simulink model "scara_ctc_sim"  (R2024a)
settings: Solver=ode4  StartTime=0.0  StopTime=4.0  FixedStep=0.005  RelTol=1e-3
settings Model: Creator=42962  LastModifiedBy=42962

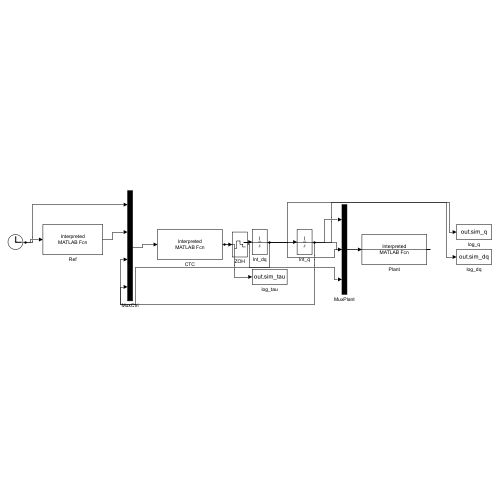
[thumbnail: Simulink's stored preview of the top-level diagram]
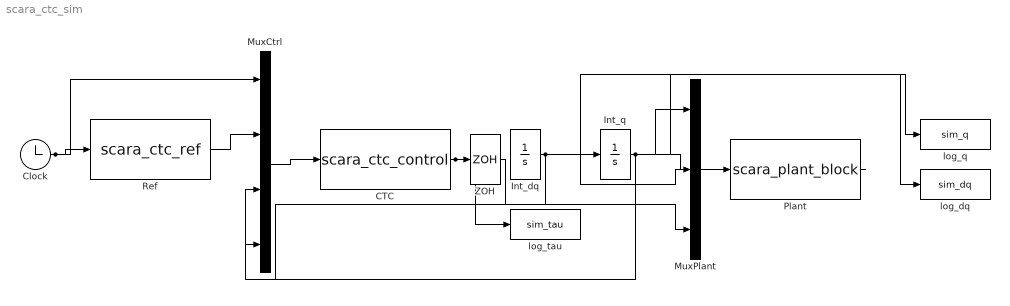
== system scara_ctc_sim ==
  CTC : MATLABFcn  MATLABFcn=scara_ctc_control  OutputDimensions=4
  Clock : Clock
  Int_dq : Integrator  InitialCondition=zeros(4,1)
  Int_q : Integrator  InitialCondition=[0;0;0.05;0]
  MuxCtrl : Mux
  MuxPlant : Mux  Inputs=3
  Plant : MATLABFcn  MATLABFcn=scara_plant_block  OutputDimensions=4
  Ref : MATLABFcn  MATLABFcn=scara_ctc_ref  OutputDimensions=12
  ZOH : ZeroOrderHold  SampleTime=0.005
  log_dq : ToWorkspace  VariableName=sim_dq  SaveFormat=Structure With Time  SampleTime=-1
  log_q : ToWorkspace  VariableName=sim_q  SaveFormat=Structure With Time  SampleTime=-1
  log_tau : ToWorkspace  VariableName=sim_tau  SaveFormat=Structure With Time  SampleTime=-1
  wires:
  Clock/1 -> Ref/1, MuxCtrl/1
  Ref/1 -> MuxCtrl/2
  Int_q/1 -> MuxCtrl/3, MuxPlant/1, log_q/1
  Int_dq/1 -> MuxCtrl/4, Int_q/1, MuxPlant/2, log_dq/1
  MuxCtrl/1 -> CTC/1
  CTC/1 -> ZOH/1, log_tau/1
  ZOH/1 -> MuxPlant/3
  MuxPlant/1 -> Plant/1
  Plant/1 -> Int_dq/1
